simulink model "Battery_Model_First_Order"  (R2025b)
settings: Solver=ode23t  StartTime=0.0  StopTime=500  MaxStep=0.1  RelTol=1e-3  AbsTol=1e-6
libraries: fl_lib x8, nesl_utility x6, simulink x1
settings Model: Creator=psvan  LastModifiedBy=psvan

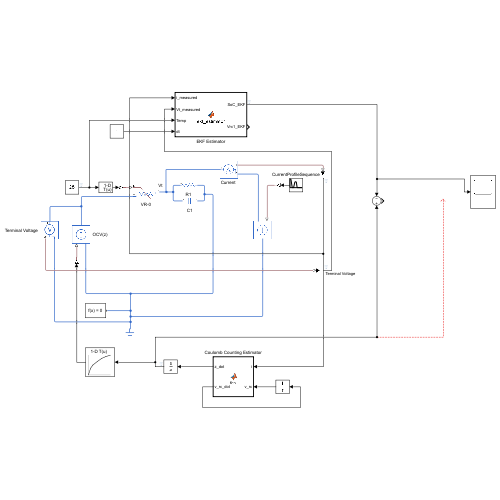
[thumbnail: Simulink's stored preview of the top-level diagram]
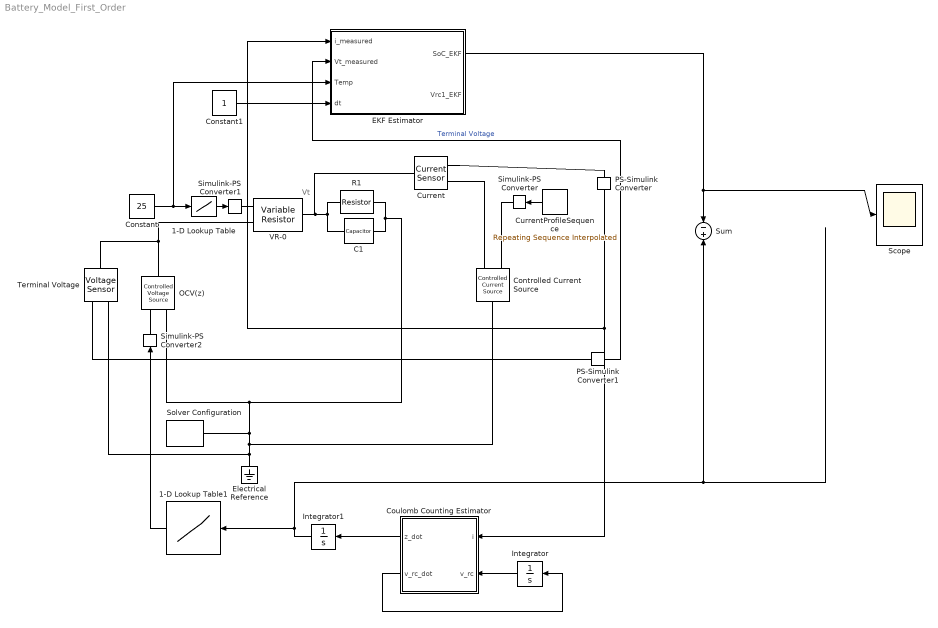
== system Battery_Model_First_Order ==
  note: Vt
  1-D Lookup Table : Lookup_n-D  NumberOfTableDimensions=1  BreakpointsForDimension1=[0, 25, 40]  Table=[0.019, 0.02, 0.021]  ExtrapMethod=Clip  InternalRulePriority=Speed  RndMeth=Simplest
  1-D Lookup Table1 : Lookup_n-D  NumberOfTableDimensions=1  BreakpointsForDimension1=[0 0.1 0.2 0.4 0.6 0.8 1]  Table=[3.0 3.4 3.6 3.8 4.0 4.1 4.2]  InternalRulePriority=Speed  RndMeth=Simplest
  C1 : fl_lib/Electrical/Electrical Elements/Capacitor  c=500 F  r=1e-6 Ohm  g=0 1/Ohm  i_specify=off  i_priority=None  i=0 A  i_nominal_specify=off  i_nominal_value=1  i_nominal_unit=A  v_specify=off  v_priority=None  v=0 V  v_nominal_specify=off  v_nominal_value=1  v_nominal_unit=V  vc_specify=off  vc_priority=High  vc=0 V  vc_nominal_specify=off  vc_nominal_value=1  vc_nominal_unit=V
  Constant : Constant  Value=25
  Constant1 : Constant
  Controlled Current Source : fl_lib/Electrical/Electrical Sources/Controlled Current Source
  Coulomb Counting Estimator : MATLAB Function  TreatAsAtomicUnit=on
  "Current " : fl_lib/Electrical/Electrical Sensors/Current Sensor
  CurrentProfileSequence : simulink/Sources/Repeating Sequence Interpolated  OutValues=[15 15 0 0 10 10 0 0]  TimeValues=[0 50 100 150 200 250 300 500]  LookUpMeth=Interpolation-Use End Values  tsamp=0.01  OutMin=[]  OutMax=[]  OutDataTypeStr=double  OutputDataTypeScalingMode=double  OutDataType=fixdt(0,8)  OutScaling=2^-10
  EKF Estimator : MATLAB Function  TreatAsAtomicUnit=on  SystemSampleTime=1
  Electrical Reference : fl_lib/Electrical/Electrical Elements/Electrical Reference
  Integrator : Integrator
  Integrator1 : Integrator  InitialCondition=0.5
  OCV(z) : fl_lib/Electrical/Electrical Sources/Controlled Voltage Source
  PS-Simulink Converter : nesl_utility/PS-Simulink Converter  PhysicalDomain=network_engine_domain  SubClassName=ps_output  LeftPortType=input  RightPortType=output  PseudoPeriodic=off  Frequencies=[]  VectorFormat=inherit  Unit=inherit  AffineConversion=off
  PS-Simulink Converter1 : nesl_utility/PS-Simulink Converter  PhysicalDomain=network_engine_domain  SubClassName=ps_output  LeftPortType=input  RightPortType=output  PseudoPeriodic=off  Frequencies=[]  VectorFormat=inherit  Unit=inherit  AffineConversion=off
  R1 : fl_lib/Electrical/Electrical Elements/Resistor  R=0.01 Ohm  i_specify=off  i_priority=None  i=0 A  i_nominal_specify=off  i_nominal_value=1  i_nominal_unit=A  v_specify=off  v_priority=None  v=0 V  v_nominal_specify=off  v_nominal_value=1  v_nominal_unit=V
  Scope : Scope
      settings: ActiveDisplayYMinimum=-4.1392968767523648  ActiveDisplayYMaximum=15.226471411955179
  Simulink-PS Converter : nesl_utility/Simulink-PS Converter  PhysicalDomain=network_engine_domain  SubClassName=ps_input  LeftPortType=input  RightPortType=output  PseudoPeriodic=off  Frequencies=[]  NoiseDistribution=none  NoiseParameters=[]  Unit=1  AffineConversion=off  FilteringAndDerivatives=provide  SimscapeFilterOrder=1  InputFilterTimeConstant=0.001  UdotUserProvided=0
  Simulink-PS Converter1 : nesl_utility/Simulink-PS Converter  PhysicalDomain=network_engine_domain  SubClassName=ps_input  LeftPortType=input  RightPortType=output  PseudoPeriodic=off  Frequencies=[]  NoiseDistribution=none  NoiseParameters=[]  Unit=1  AffineConversion=off  FilteringAndDerivatives=provide  SimscapeFilterOrder=1  InputFilterTimeConstant=0.001  UdotUserProvided=0
  Simulink-PS Converter2 : nesl_utility/Simulink-PS Converter  PhysicalDomain=network_engine_domain  SubClassName=ps_input  LeftPortType=input  RightPortType=output  PseudoPeriodic=off  Frequencies=[]  NoiseDistribution=none  NoiseParameters=[]  Unit=1  AffineConversion=off  FilteringAndDerivatives=provide  SimscapeFilterOrder=1  InputFilterTimeConstant=0.001  UdotUserProvided=0
  Solver Configuration : nesl_utility/Solver Configuration  PhysicalDomain=network_engine_domain  SubClassName=solver  LeftPortType=input  RightPortType=generic  Tones=[]  Harmonics=[]  SimulateNoise=off  Profile=off  UseLocalSampling=off  EnableSwitchedLinearOptims=on  FrequencyDomain=off  UseCCode=off  RelTol=0.001  AbsTol=0.001  MinStep=1e-09  ToWorkspace=off  RevertToSquareIcSolve=off  NumHomotopyIterations=100  PhasorMode=off  PhasorModeNumHarmonics=1  ConsistencySolver=NEWTON_XTOL_AFTER_FTOL  IndexReductionMethod=DerivativeReplacement  DoDC=off  ResidualTolerance=1e-09  ConsistencyTolSource=GLOBAL  ConsistencyAbsTol=0.001  ConsistencyRelTol=0.001  ConsistencyTolFactor=0.001  UseLocalSolver=off  LocalSolverChoice=NE_BACKWARD_EULER_ADVANCER  ResolveIndetEquations=on  FunctionEvalNumThread=1  LocalSolverSampleTime=0.001  DoFixedCost=off  MaxNonlinIter=3  MaxModeIter=2  ComputeImpulses=off  ImpulseIterations=2  LinearAlgebra=auto  LinearAlgebraNumThread=0  EquationFormulation=NE_TIME_EF  DelaysMemoryBudget=1024  AutomaticFiltering=on  FilteringTimeConstant=0.001  PartitionStorageMethod=AS_NEEDED  PartitionMemoryBudget=1024  PartitionMethod=ROBUST  MultibodyUseLocalSolver=off  MultibodyLocalSolverChoice=ODE1  MultibodyLocalSolverSampleTime=0.001
  Sum : Sum  Inputs=-+
  Terminal Voltage : fl_lib/Electrical/Electrical Sensors/Voltage Sensor
  VR-0 : fl_lib/Electrical/Electrical Elements/Variable Resistor  Rmin=0.02 Ohm  thermalEnable=false  thermal_mass=1 J/K  i_specify=off  i_priority=None  i=0 A  i_nominal_specify=off  i_nominal_value=1  i_nominal_unit=A  v_specify=off  v_priority=None  v=0 V  v_nominal_specify=off  v_nominal_value=1  v_nominal_unit=V  T_specify=off  T_priority=None  T=300 K  T_nominal_specify=off  T_nominal_value=1  T_nominal_unit=K
  wires:
  Constant/1 -> EKF Estimator/3(Temp), 1-D Lookup Table/1
  1-D Lookup Table/1 -> Simulink-PS Converter1/1
  Integrator/1 -> Coulomb Counting Estimator/2(v_rc)
  Coulomb Counting Estimator/2(v_rc_dot) -> Integrator/1
  Coulomb Counting Estimator/1(z_dot) -> Integrator1/1
  CurrentProfileSequence/1 -> Simulink-PS Converter/1
  Integrator1/1 -> Sum/2, 1-D Lookup Table1/1
  1-D Lookup Table1/1 -> Simulink-PS Converter2/1
  PS-Simulink Converter/1 -> EKF Estimator/1(i_measured), Coulomb Counting Estimator/1(i)
  PS-Simulink Converter1/1 -> EKF Estimator/2(Vt_measured)  "Terminal Voltage"
  Constant1/1 -> EKF Estimator/4(dt)
  EKF Estimator/1(SoC_EKF) -> Sum/1, Scope/1
  connections:
  OCV(z)/LConn1 -- Terminal Voltage/LConn1 -- VR-0/LConn2
  C1/LConn1 -- "Current "/LConn1 -- VR-0/RConn1 -- R1/LConn1
  C1/RConn1 -- OCV(z)/RConn2 -- Solver Configuration/RConn1 -- Controlled Current Source/LConn1 -- Terminal Voltage/RConn2 -- Electrical Reference/LConn1 -- R1/RConn1
  Simulink-PS Converter1/RConn1 -- VR-0/LConn1
  Simulink-PS Converter2/RConn1 -- OCV(z)/RConn1
  "Current "/RConn1 -- PS-Simulink Converter/LConn1
  PS-Simulink Converter1/LConn1 -- Terminal Voltage/RConn1
  Controlled Current Source/RConn2 -- "Current "/RConn2
  Simulink-PS Converter/RConn1 -- Controlled Current Source/RConn1

== matlab function Battery_Model_First_Order/EKF Estimator ==
  data: i_measured input; SoC_EKF output; Vt_measured input; Temp input; dt input; Vrc1_EKF output
function [SoC_EKF, Vrc1_EKF] = ekf_estimator(i_measured, Vt_measured, Temp, dt)

persistent x_hat P is_initialized;

Q = 3600;      
eta = 0.995;   
R1 = 0.01;     
C1 = 500;      
tau1 = R1 * C1; 
soc_bp = [0, 0.1, 0.2, 0.4, 0.6, 0.8, 1];
ocv_lut = [3.0, 3.4, 3.6, 3.8, 4.0, 4.1, 4.2]; % OCV values (V)
temp_bp = [0, 25, 40];
R0_lut = [0.019, 0.02, 0.021]; 

Q_mat = diag([1e-7, 1e-5]);

R_mat = 1e-1; 


if isempty(is_initialized) || dt <= 0 
    x_hat = [0.5; 0]; 

    P = diag([1e-3, 0.1]); 
    is_initialized = true;
    fprintf('EKF Initialized.\n');
end

soc_prev = x_hat(1);
vrc1_prev = x_hat(2);
i_prev = i_measured; 

soc_pred = soc_prev - (eta * dt / Q) * i_prev;
vrc1_pred = vrc1_prev * exp(-dt / tau1) + R1 * (1 - exp(-dt / tau1)) * i_prev;
x_pred = [soc_pred; vrc1_pred]; 

A = zeros(2, 2);
A(1,1) = 1;                     
A(1,2) = 0;                     
A(2,1) = 0;                     
A(2,2) = exp(-dt / tau1);      

% Predict covariance P(k|k-1)
P_pred = A * P * A' + Q_mat;

% --- Update Step ---
% Use predicted state for calculations at time k
soc_pred_k = x_pred(1);
vrc1_pred_k = x_pred(2);
i_k = i_measured; 
temp_k = Temp;    

soc_pred_k_clamped = max(soc_bp(1)+eps, min(soc_bp(end)-eps, soc_pred_k));

ocv_pred = interp1(soc_bp, ocv_lut, soc_pred_k_clamped, 'linear');

delta_soc = 0.001; 
ocv_plus = interp1(soc_bp, ocv_lut, soc_pred_k_clamped + delta_soc, 'linear', 'extrap');
ocv_minus = interp1(soc_bp, ocv_lut, soc_pred_k_clamped - delta_soc, 'linear', 'extrap');
dOCV_dz = (ocv_plus - ocv_minus) / (2 * delta_soc);
if isnan(dOCV_dz) || isinf(dOCV_dz)
    dOCV_dz = (interp1(soc_bp, ocv_lut, soc_bp(2)) - interp1(soc_bp, ocv_lut, soc_bp(1))) / (soc_bp(2) - soc_bp(1)); % Use slope at start
    if soc_pred_k_clamped > soc_bp(end-1)
         dOCV_dz = (interp1(soc_bp, ocv_lut, soc_bp(end)) - interp1(soc_bp, ocv_lut, soc_bp(end-1))) / (soc_bp(end) - soc_bp(end-1)); % Use slope at end
    end
    if isnan(dOCV_dz), dOCV_dz = 0; end % Final fallback
end

R0_k = interp1(temp_bp, R0_lut, temp_k, 'linear', 'extrap');

Vt_pred = ocv_pred - vrc1_pred_k - i_k * R0_k;

C = zeros(1, 2);
C(1,1) = dOCV_dz; 
C(1,2) = -1;      

Innovation_cov = C * P_pred * C' + R_mat;
K = P_pred * C' / Innovation_cov; 

x_hat = x_pred + K * (Vt_measured - Vt_pred);

P = (eye(2) - K * C) * P_pred;

P = (P + P') / 2;

SoC_EKF = x_hat(1);
SoC_EKF = max(0, min(1, SoC_EKF));

Vrc1_EKF = x_hat(2);

end

== matlab function Battery_Model_First_Order/Coulomb Counting Estimator ==
  data: i input; z_dot output; v_rc input; v_rc_dot output
function [z_dot, v_rc_dot] = fcn(i, v_rc)
Q = 3600;
eta = 0.995;
R1 = 0.01;
C1 = 500;
z_dot = -(eta * i) / Q; 
v_rc_dot = (i / C1) - (v_rc / (R1 * C1));
end
